simulink model "ControladorTraslacionPID"  (R2026b)
settings: Solver=VariableStepAuto
settings Model: Creator=fedeb  LastModifiedBy=fedeb

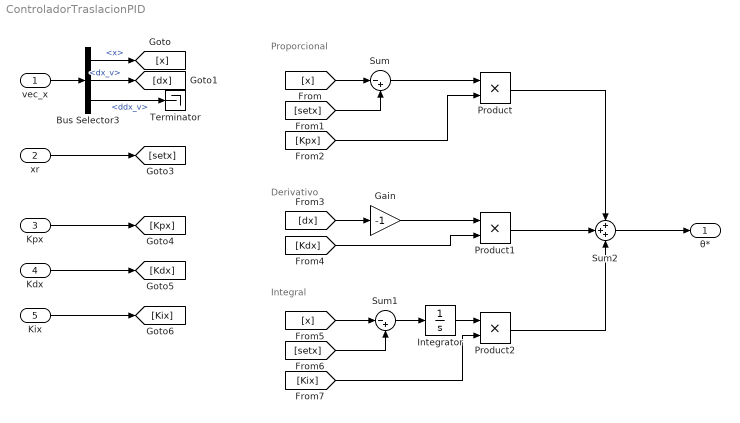
== system ControladorTraslacionPID ==
  note: Proporcional
  note: Integral
  note: Derivativo
  vec_x : Inport
  xr : Inport  Port=2
  Kpx : Inport  Port=3
  Kdx : Inport  Port=4
  Kix : Inport  Port=5
  Bus Selector3 : BusSelector  OutputSignals=x,dx_v,ddx_v
  Gain : Gain  Gain=-1
  Integrator : Integrator
  Product : Product
  Product1 : Product
  Product2 : Product
  Sum : Sum  Inputs=|-+
  Sum1 : Sum  Inputs=|-+
  Sum2 : Sum  Inputs=+++
  Terminator : Terminator
  θ* : Outport
  wires:
  xr/1 -> [setx]
  Product2/1 -> Sum2/3
  Sum2/1 -> θ*/1
  Sum1/1 -> Integrator/1
  [setx] -> Sum1/2
  [x] -> Sum1/1
  Product/1 -> Sum2/1
  Product1/1 -> Sum2/2
  [Kix] -> Product2/2
  Gain/1 -> Product1/1
  Integrator/1 -> Product2/1
  [dx] -> Gain/1
  [Kdx] -> Product1/2
  [x] -> Sum/1
  [Kpx] -> Product/2
  [setx] -> Sum/2
  Sum/1 -> Product/1
  vec_x/1 -> Bus Selector3/1
  Bus Selector3/1 -> [x]  "<x>"
  Bus Selector3/2 -> [dx]  "<dx_v>"
  Bus Selector3/3 -> Terminator/1  "<ddx_v>"
  Kix/1 -> [Kix]
  Kdx/1 -> [Kdx]
  Kpx/1 -> [Kpx]
